simulink model "ASM_Traffic"  (R2026a)
settings: Solver=ode1  StartTime=SIM.tstart.v  StopTime=SIM.tend.v  FixedStep=SIM.StepSize.v
PostLoadFcn:
  | if any(exist('dsrtsu_mdlpostloadfcn', 'file') ~= 0), dsrtsu_mdlpostloadfcn('Execute', bdroot); end
  | try, asm_mdl_postloadfcn(bdroot, 'UpdateModel', 3600); catch, disp(lasterr); end,
InitFcn:
  | , if any(exist('rtifpga_mdlclblib', 'file') ~= 0), rtifpga_mdlclblib('Init', bdroot); end,
  | , if any(exist('dsmpb_private', 'file') ~= 0), dsmpb_private('dsmpb_mdlclblib', 'Init', bdroot); end,
model workspace (MAT data in the model file):
  asmReferencePath = [0 0.01 0.02 0.03 0.04 0.05 0.06 0.07 0.08 0.09 0.1 0.11 ... (350007 elements, 50001x7)]
  roadBounds : Simulink.Parameter (value not decoded)
  safetyAxes : Simulink.Parameter (value not decoded)
undefined symbols (not defined in the file): _to_, a0b2, ASM_BrakeHydraulics_DemoSystems, ASM_VehicleDynamics_DemoSystems, b98103fe8ad365046cd0, BrakeCircuit, controllerConfig, CPT, Crankshaft, DiscIntNeverNeededParam, dsmsi, FinalDriveAssembly, MDL, ModeSignals, mu, Pos_BrakePedal_Maneuver, rad, RefSignals, roadFamilyData, roadFamilyId, s_to_rpm, SIM, SoftECU, Suspension, Tire, Transmission
libraries: ASM_Traffic_lib x135, simulink x98, ASM_Utils_lib x77, ASM_VehicleDynamics_lib x70, ASM_Environment_lib x22, dsmpblib x20, dsmsilib x15, MDLD_Utils_lib x10, ASM_BrakeHydraulics_lib x3, sl_discontinuities x2
(part 23 of 65)

== system ASM_Traffic/Drivetrain/Plant/Drivetrain/Transmission ==
  n_Engine[rad|s] : Inport
  Reset[0|1] : Inport  Port=2
  Trq_Engine[Nm] : Inport  Port=3
  Mode_Transmission[1|2] : Inport  Port=4
  Pos_ClutchPedal_MT[%] : Inport  Port=5
  Gear_MT[] : Inport  Port=6
  Enable_v_Init[0|1] : Inport  Port=7
  ECU_Signals : Inport  Port=8
  omega_In_Diff[rad|s] : Inport  Port=9
  ASMSignalCollector : Subsystem
  AutomaticActive : simulink/Logic and Bit Operations/Compare To Constant  relop===  const=2  OutDataTypeStr=boolean
  AutomaticTransmission : Subsystem  TreatAsAtomicUnit=on
  Bus Selector2 : BusSelector  OutputSignals=Ctrl_Lockup_Clutch[0_1],Gear[]
  Dummy : Constant  Value=0
  Goto Tag Visibility1 : GotoTagVisibility  GotoTag=ASMBUS_ManualTransmission
  Goto Tag Visibility2 : GotoTagVisibility  GotoTag=ASMBUS_AutomaticTransmission
  ManualActive : simulink/Logic and Bit Operations/Compare To Constant  relop===  const=1  OutDataTypeStr=boolean
  ManualTransmission : Subsystem  TreatAsAtomicUnit=on
  Multiport Switch : MultiPortSwitch  Inputs=2  InputSameDT=off
  Multiport Switch1 : MultiPortSwitch  Inputs=2  InputSameDT=off
  Multiport Switch2 : MultiPortSwitch  Inputs=2  InputSameDT=off
  Sat_TrmMode : Saturate  UpperLimit=2  LowerLimit=1
  Terminator : Terminator
  Trq_Fric[Nm] : Outport  VectorParamsAs1DForOutWhenUnconnected=off
  omega_In_Trm[rad|s] : Outport  Port=2  VectorParamsAs1DForOutWhenUnconnected=off
  Inertia_Out_Trm[kgm2] : Outport  Port=3  VectorParamsAs1DForOutWhenUnconnected=off
  Trq_Out_Trm[Nm] : Outport  Port=4  VectorParamsAs1DForOutWhenUnconnected=off
  tag scope: ASMBUS_AutomaticTransmission=scoped, ASMBUS_ManualTransmission=scoped
  wires:
  AutomaticTransmission/3(omega_In_Trm[rad|s]) -> Multiport Switch2/3
  Multiport Switch2/1 -> omega_In_Trm[rad|s]/1
  ManualTransmission/3(omega_In_Trm[rad|s]) -> Multiport Switch2/2
  Enable_v_Init[0|1]/1 -> ManualTransmission/6(Enable_v_Init[0|1]), AutomaticTransmission/6(Enable_v_Init[0|1])
  n_Engine[rad|s]/1 -> ManualTransmission/3(n_Engine[rad|s]), AutomaticTransmission/3(n_Engine[rad|s])
  ECU_Signals/1 -> Bus Selector2/1
  ManualTransmission/1(ASMSignalBus) -> [ASMBUS_ManualTransmission]
  AutomaticTransmission/1(ASMSignalBus) -> [ASMBUS_AutomaticTransmission]
  Bus Selector2/2 -> ASMSignalCollector/3(Gear_AT[]), AutomaticTransmission/2(Gear[])  "<Gear[]>"
  Bus Selector2/1 -> AutomaticTransmission/1(Ctrl_Lockup_Clutch[0_1])  "<Ctrl_Lockup_Clutch[0_1]>"
  Sat_TrmMode/1 -> AutomaticActive/1, ManualActive/1, Multiport Switch/1, Multiport Switch1/1, ASMSignalCollector/1(Mode_Transmission[1|2]), Multiport Switch2/1
  ManualActive/1 -> ManualTransmission/Enable
  Trq_Engine[Nm]/1 -> Terminator/1
  Reset[0|1]/1 -> ManualTransmission/5(Reset[0|1]), AutomaticTransmission/5(Reset[0|1])
  AutomaticTransmission/4(Trq_Out_Trm[Nm]) -> Multiport Switch1/3
  AutomaticTransmission/2(Trq_In_Converter[Nm]) -> Multiport Switch/3
  Multiport Switch1/1 -> Trq_Out_Trm[Nm]/1
  Multiport Switch/1 -> Trq_Fric[Nm]/1
  Dummy/1 -> Inertia_Out_Trm[kgm2]/1
  ManualTransmission/2(Trq_Fric[Nm]) -> Multiport Switch/2
  ManualTransmission/4(Trq_Out_Trm[Nm]) -> Multiport Switch1/2
  Mode_Transmission[1|2]/1 -> Sat_TrmMode/1
  Pos_ClutchPedal_MT[%]/1 -> ManualTransmission/1(Pos_ClutchPedal[%])
  Gear_MT[]/1 -> ASMSignalCollector/2(Gear_MT[]), ManualTransmission/2(Gear[])
  omega_In_Diff[rad|s]/1 -> ManualTransmission/4(omega_In_Diff[rad|s]), AutomaticTransmission/4(omega_In_Diff[rad|s])
  AutomaticActive/1 -> AutomaticTransmission/Enable

== system ASM_Traffic/Drivetrain/Plant/UserInterface/ASMSignalBus_Plant ==
  In : Inport
  Terminator_1 : Terminator
  tag scope: ASMBUS_Drivetrain_Plant=global
  wires:
  In/1 -> [ASMBUS_Drivetrain_Plant]  "Plant"
  [ASMBUS_Drivetrain_Plant] -> Terminator_1/1

== system ASM_Traffic/Drivetrain/Plant/UserInterface/DISP_Plant ==
  In : Inport
  ActiveTransmission : Subsystem
  AutomaticTransmission : Subsystem
  Bus Selector2 : BusSelector  OutputSignals=Crankshaft,Starter,FinalDriveAssembly.Shaft_CF.Trq_CF_Shaft[Nm],FinalDriveAssembly.Shaft_CR.Trq_CR_Shaft[Nm],FinalDriveAssembly.Shaft_FL.Trq_FL_Shaft[Nm],FinalDriveAssembly.Shaft_FR.Trq_FR_Shaft[Nm],FinalDriveAssembly.Shaft_RL.Trq_RL_Shaft[Nm],FinalDriveAssembly.Shaft_RR.Trq_RR_Shaft[Nm],Transmission.OutputSignals,Transmission.Manual,Transmission.Automatic
  EngineSpeed : Subsystem
  ManualTransmission : Subsystem
  Shafts : Subsystem
  wires:
  In/1 -> Bus Selector2/1
  Bus Selector2/7 -> Shafts/5(Shaft_RL)  "<Trq_RL_Shaft[Nm]>"
  Bus Selector2/1 -> EngineSpeed/1(Crankshaft)  "<Crankshaft>"
  Bus Selector2/10 -> ManualTransmission/1(ManTrm)  "<Manual>"
  Bus Selector2/2 -> EngineSpeed/2(Starter)  "<Starter>"
  Bus Selector2/4 -> Shafts/2(Shaft_CR)  "<Trq_CR_Shaft[Nm]>"
  Bus Selector2/3 -> Shafts/1(Shaft_CF)  "<Trq_CF_Shaft[Nm]>"
  Bus Selector2/9 -> ActiveTransmission/1(ActiveTrm)  "<OutputSignals>"
  Bus Selector2/6 -> Shafts/4(Shaft_FR)  "<Trq_FR_Shaft[Nm]>"
  Bus Selector2/5 -> Shafts/3(Shaft_FL)  "<Trq_FL_Shaft[Nm]>"
  Bus Selector2/8 -> Shafts/6(Shaft_RR)  "<Trq_RR_Shaft[Nm]>"
  Bus Selector2/11 -> AutomaticTransmission/1(AutoTrm)  "<Automatic>"

== system ASM_Traffic/Drivetrain/Plant/UserInterface/PAR_Plant ==
  Bus Creator1 : BusCreator  Inputs=5
  Const_LoadTorque[Nm] : Constant  Value=0
  DRIVETRAIN_VARIANT_SWITCHES : ASM_VehicleDynamics_lib/Drivetrain/DRIVETRAIN_VARIANT_SWITCHES  Tag=ASM_SUBCOMPONENT  SW_Transmission_Mode=MDL.Drivetrain.SW_Transmission_Mode.v  SW_Drivetrain_Mode=MDL.Drivetrain.SW_Drivetrain_Mode.v  ASMProperties=struct('Name','DRIVETRAIN_VARIANT_SWITCHES','Version','5.0','Library','ASM_VehicleDynamics_lib')  ASMInstanceName=drivetrain_variant_switches  ASMInstanceID=1
  ModelDesk_MC_ID_Drivetrain : ASM_Utils_lib/ModelDeskInterface/ModelDesk_MC  Tag=ASM_MAINCOMPONENT  Editable=off  MainComponent=Drivetrain
  Sw_CrankShaft_Reset[0Disabled|1Enabled] : Constant
  Sw_LoadTorque[0Clutch|1Constant] : Constant  Value=0
  Out : Outport  VectorParamsAs1DForOutWhenUnconnected=off
  wires:
  Sw_LoadTorque[0Clutch|1Constant]/1 -> Bus Creator1/3  "Sw_LoadTorque[0Clutch|1Constant]"
  Const_LoadTorque[Nm]/1 -> Bus Creator1/4  "Const_LoadTorque[Nm]"
  Sw_CrankShaft_Reset[0Disabled|1Enabled]/1 -> Bus Creator1/5  "Sw_CrankShaft_Reset[0Disabled|1Enabled]"
  DRIVETRAIN_VARIANT_SWITCHES/2 -> Bus Creator1/2  "Mode_Drivetrain[1AWD|2FWD|3RWD|4FF-4WD|5FF]"
  Bus Creator1/1 -> Out/1  "UserInterface"
  DRIVETRAIN_VARIANT_SWITCHES/1 -> Bus Creator1/1  "Mode_Transmission[1Manual|2Automatic]"

== system ASM_Traffic/Drivetrain/SignalInterface/ASMSignalInterface/signal_structure ==
  ASMSignalBus : Inport
  Automatic : BusSelector  OutputSignals=LockUpClutch,GearBox,TorqueConverter
  BusSelector_1 : BusSelector  OutputSignals=Control,Plant
  CentralDifferential : BusSelector  OutputSignals=omega_Cage[rad|s],omega_In_CentralDiff[rad|s],Shaft_CF,Shaft_CR,Trq_Lock[Nm],omega_Out_Front_CentralDiff[rad|s],omega_Out_Rear_CentralDiff[rad|s],Const_i_MainReductionGear[],Const_TrqDistribution[]
  Clutch : BusSelector  OutputSignals=Trq_Fric_Clutch[Nm],omega_delta_Clutch[rad|s],omega_Out_ClutchPlate[rad|s],Trq_TorsionSpring_Clutch[Nm]
  Clutch_4WD : BusSelector  OutputSignals=omega_Clutch_4WD_In[rad|s],Trq_Lock_Clutch_4WD[Nm],omega_Clutch_4WD_Out[rad|s]
  ContentID : Constant  Value=632359247
  Control : BusSelector  OutputSignals=Lockup_Clutch_Control,Shift_Lock_Control,Shift_Strategy,Tip_Shift_Control,Torque_Intervention_Control
  Crankshaft : BusSelector  OutputSignals=Trq_Mass_Mod[Nm],Const_Inertia_Engine[kgm2],Trq_Eff_Crank[Nm],n_Engine[rad|s],n_Engine[rpm]
  FinalDriveAssembly : BusSelector  OutputSignals=i_FrontDrive[],i_RearDrive[],TrqDistri_Front_Rear[0_1],i_FinalDrive[],CentralDifferential,FrontDifferential,RearDifferential,Shaft_TGCL4WD,Shaft_CF,Shaft_CR,TransferGearbox,Clutch_4WD,Shaft_FL,Shaft_FR,Shaft_RL,Shaft_RR,Trq_Out_Front_Diff[Nm],Trq_Shaft[FL;FR;RL;RR][Nm]
  FrontDifferential : BusSelector  OutputSignals=omega_Cage[rad|s],omega_In_FrontDifferential[rad|s],Shaft_FL,Shaft_FR,Trq_Lock_FrontDifferential[Nm],omega_Out_Left_FrontDifferential[rad|s],omega_Out_Right_FrontDifferential[rad|s],Const_i_MainReductionGear[],Const_TrqDistribution[]
  GearBox : BusSelector  OutputSignals=i_unsync_Trm[],i_Trm[],Trq_Out_Trm[Nm],omega_In_Trm[rad|s],omega_Out_Trm[rad|s],Inertia_Trm[kgm2]
  GearBox1 : BusSelector  OutputSignals=i_unsync_Trm[],i_Trm[],Trq_Out_Trm[Nm],omega_In_Trm[rad|s],omega_Out_Trm[rad|s],Inertia_Trm[kgm2]
  InfoBlock : Subsystem
      mask Display: fprintf('Structural changes of the signal bus require an update \nof the ''ASMSignalCollector'' block. \n\nTo start the update process double click the parent block.\n\n WARNING:\n During update this subsystem will be cleared completely')
  LockUpClutch : BusSelector  OutputSignals=Trq_Fric_Clutch[Nm],omega_delta_Clutch[rad|s],omega_Out_ClutchPlate[rad|s],Trq_TorsionSpring_Clutch[Nm]
  Lockup_Clutch_Control : BusSelector  OutputSignals=Ctrl_Lockup_Clutch[0_1]
  MDLD_DATA_CAPTURE : MDLD_Utils_lib/ModelDeskPlotInterface/DataCapture_Sfcn/MDLD_DATA_CAPTURE  inputPortWidth=94  measurementSignals=[0 0 0 0 0 0 0 0 0 0 0 0 0 0 0 0 0 0 0 0 0 0 0 0 0 0 0 0 0 0 0 0 0 0 0 0 0 0 0 0 0 0 0 0 0 0 0 0 0 0 0 0 0 0 0 0 0 0 0 0 0 0 0 0 0 0 0 0 0 0 0 0 0 0 0 0 0 0 0 0 0 0 0 0 0 0 0 0 0 0 0 0 0 0]  downsampling=1  samplingPeriod=SIM.StepSize.v  uuid=0  ASMProperties=struct('Name','mdld_data_capture','Version','1.0','Library','mdld_utils_lib')  startTriggerDelay=0  startTriggerLogic=0  startTriggerCount=0  startTriggerConditions=[0,0,0,0,0,0,0,0,0]  stopTriggerDelay=0  stopTriggerLogic=0  stopTriggerCount=0  stopTriggerConditions=[0,0,0,0,0,0,0,0,0]  ContentID_RefStruct=632359247
  Manual : BusSelector  OutputSignals=Clutch,GearBox
  OutputSignals : BusSelector  OutputSignals=i_unsync_Trm[],i_Trm[],Trq_Out_Trm[Nm],omega_In_Trm[rad|s],Inertia_Trm[kgm2],omega_Out_Trm[rad|s],Gear[]
  Plant : BusSelector  OutputSignals=Crankshaft,Starter,TestBench,Transmission,FinalDriveAssembly,Type_Engine_1[0Unkown|1Other|2Otto|3Diesel|4Electric],Trq_MeanEff_Engine[Nm]
  RearDifferential : BusSelector  OutputSignals=omega_Cage[rad|s],omega_In_RearDifferential[rad|s],Shaft_RL,Shaft_RR,Trq_Lock_RearDifferential[Nm],omega_Out_Left_RearDifferential[rad|s],omega_Out_Right_RearDifferential[rad|s],Const_i_MainReductionGear[],Const_TrqDistribution[]
  Reshape_89 : Reshape
  Shaft_CF : BusSelector  OutputSignals=Trq_CF_Shaft[Nm]
  Shaft_CF1 : BusSelector  OutputSignals=Trq_CF_Shaft[Nm]
  Shaft_CR : BusSelector  OutputSignals=Trq_CR_Shaft[Nm]
  Shaft_CR1 : BusSelector  OutputSignals=Trq_CR_Shaft[Nm]
  Shaft_FL : BusSelector  OutputSignals=Trq_FL_Shaft[Nm]
  Shaft_FL1 : BusSelector  OutputSignals=Trq_FL_Shaft[Nm]
  Shaft_FR : BusSelector  OutputSignals=Trq_FR_Shaft[Nm]
  Shaft_FR1 : BusSelector  OutputSignals=Trq_FR_Shaft[Nm]
  Shaft_RL : BusSelector  OutputSignals=Trq_RL_Shaft[Nm]
  Shaft_RL1 : BusSelector  OutputSignals=Trq_RL_Shaft[Nm]
  Shaft_RR : BusSelector  OutputSignals=Trq_RR_Shaft[Nm]
  Shaft_RR1 : BusSelector  OutputSignals=Trq_RR_Shaft[Nm]
  Shaft_TGCL4WD : BusSelector  OutputSignals=Trq_TGCL4WD_Shaft[Nm]
  Shift_Lock_Control : BusSelector  OutputSignals=Ctrl_Parking_Pawl[0|1]
  Shift_Strategy : BusSelector  OutputSignals=Gear_Requested[]
  SignalFilter : Mux  Inputs=91
  SignalFilterGain : Gain
  Starter : BusSelector  OutputSignals=Trq_Starter[Nm],Inertia_Starter[kgm2]
  Terminator : Terminator
  TestBench : BusSelector  OutputSignals=Trq_TestBench[Nm],Inertia_TestBench[kgm2]
  Tip_Shift_Control : BusSelector  OutputSignals=Gear_Requested[]
  TorqueConverter : BusSelector  OutputSignals=Trq_Pump[Nm],Trq_Turbine[Nm]
  Torque_Intervention_Control : BusSelector  OutputSignals=Factor_Trq_Engine_Red[%],Gear[]
  TransferGearbox : BusSelector  OutputSignals=Trq_Cage[Nm],omega_Shaft[rad|s]
  Transmission : BusSelector  OutputSignals=Manual,Automatic,OutputSignals
  wires:
  ASMSignalBus/1 -> BusSelector_1/1
  BusSelector_1/1 -> Control/1  "<Control>"
  Control/1 -> Lockup_Clutch_Control/1  "<Lockup_Clutch_Control>"
  Control/2 -> Shift_Lock_Control/1  "<Shift_Lock_Control>"
  Control/3 -> Shift_Strategy/1  "<Shift_Strategy>"
  Control/4 -> Tip_Shift_Control/1  "<Tip_Shift_Control>"
  Control/5 -> Torque_Intervention_Control/1  "<Torque_Intervention_Control>"
  BusSelector_1/2 -> Plant/1  "<Plant>"
  Plant/1 -> Crankshaft/1  "<Crankshaft>"
  Plant/2 -> Starter/1  "<Starter>"
  Plant/3 -> TestBench/1  "<TestBench>"
  Plant/4 -> Transmission/1  "<Transmission>"
  Transmission/1 -> Manual/1  "<Manual>"
  Manual/1 -> Clutch/1  "<Clutch>"
  Manual/2 -> GearBox/1  "<GearBox>"
  Transmission/2 -> Automatic/1  "<Automatic>"
  Automatic/1 -> LockUpClutch/1  "<LockUpClutch>"
  Automatic/2 -> GearBox1/1  "<GearBox>"
  Automatic/3 -> TorqueConverter/1  "<TorqueConverter>"
  Transmission/3 -> OutputSignals/1  "<OutputSignals>"
  Plant/5 -> FinalDriveAssembly/1  "<FinalDriveAssembly>"
  FinalDriveAssembly/5 -> CentralDifferential/1  "<CentralDifferential>"
  CentralDifferential/3 -> Shaft_CF/1  "<Shaft_CF>"
  CentralDifferential/4 -> Shaft_CR/1  "<Shaft_CR>"
  FinalDriveAssembly/6 -> FrontDifferential/1  "<FrontDifferential>"
  FrontDifferential/3 -> Shaft_FL/1  "<Shaft_FL>"
  FrontDifferential/4 -> Shaft_FR/1  "<Shaft_FR>"
  FinalDriveAssembly/7 -> RearDifferential/1  "<RearDifferential>"
  RearDifferential/3 -> Shaft_RL/1  "<Shaft_RL>"
  RearDifferential/4 -> Shaft_RR/1  "<Shaft_RR>"
  FinalDriveAssembly/8 -> Shaft_TGCL4WD/1  "<Shaft_TGCL4WD>"
  FinalDriveAssembly/9 -> Shaft_CF1/1  "<Shaft_CF>"
  FinalDriveAssembly/10 -> Shaft_CR1/1  "<Shaft_CR>"
  FinalDriveAssembly/11 -> TransferGearbox/1  "<TransferGearbox>"
  FinalDriveAssembly/12 -> Clutch_4WD/1  "<Clutch_4WD>"
  FinalDriveAssembly/13 -> Shaft_FL1/1  "<Shaft_FL>"
  FinalDriveAssembly/14 -> Shaft_FR1/1  "<Shaft_FR>"
  FinalDriveAssembly/15 -> Shaft_RL1/1  "<Shaft_RL>"
  FinalDriveAssembly/16 -> Shaft_RR1/1  "<Shaft_RR>"
  ContentID/1 -> Terminator/1
  Lockup_Clutch_Control/1 -> SignalFilter/1  "<Ctrl_Lockup_Clutch[0_1]>"
  Shift_Lock_Control/1 -> SignalFilter/2  "<Ctrl_Parking_Pawl[0|1]>"
  Shift_Strategy/1 -> SignalFilter/3  "<Gear_Requested[]>"
  Tip_Shift_Control/1 -> SignalFilter/4  "<Gear_Requested[]>"
  Torque_Intervention_Control/1 -> SignalFilter/5  "<Factor_Trq_Engine_Red[%]>"
  Torque_Intervention_Control/2 -> SignalFilter/6  "<Gear[]>"
  Crankshaft/1 -> SignalFilter/7  "<Trq_Mass_Mod[Nm]>"
  Crankshaft/2 -> SignalFilter/8  "<Const_Inertia_Engine[kgm2]>"
  Crankshaft/3 -> SignalFilter/9  "<Trq_Eff_Crank[Nm]>"
  Crankshaft/4 -> SignalFilter/10  "<n_Engine[rad|s]>"
  Crankshaft/5 -> SignalFilter/11  "<n_Engine[rpm]>"
  Starter/1 -> SignalFilter/12  "<Trq_Starter[Nm]>"
  Starter/2 -> SignalFilter/13  "<Inertia_Starter[kgm2]>"
  TestBench/1 -> SignalFilter/14  "<Trq_TestBench[Nm]>"
  TestBench/2 -> SignalFilter/15  "<Inertia_TestBench[kgm2]>"
  Clutch/1 -> SignalFilter/16  "<Trq_Fric_Clutch[Nm]>"
  Clutch/2 -> SignalFilter/17  "<omega_delta_Clutch[rad|s]>"
  Clutch/3 -> SignalFilter/18  "<omega_Out_ClutchPlate[rad|s]>"
  Clutch/4 -> SignalFilter/19  "<Trq_TorsionSpring_Clutch[Nm]>"
  GearBox/1 -> SignalFilter/20  "<i_unsync_Trm[]>"
  GearBox/2 -> SignalFilter/21  "<i_Trm[]>"
  GearBox/3 -> SignalFilter/22  "<Trq_Out_Trm[Nm]>"
  GearBox/4 -> SignalFilter/23  "<omega_In_Trm[rad|s]>"
  GearBox/5 -> SignalFilter/24  "<omega_Out_Trm[rad|s]>"
  GearBox/6 -> SignalFilter/25  "<Inertia_Trm[kgm2]>"
  LockUpClutch/1 -> SignalFilter/26  "<Trq_Fric_Clutch[Nm]>"
  LockUpClutch/2 -> SignalFilter/27  "<omega_delta_Clutch[rad|s]>"
  LockUpClutch/3 -> SignalFilter/28  "<omega_Out_ClutchPlate[rad|s]>"
  LockUpClutch/4 -> SignalFilter/29  "<Trq_TorsionSpring_Clutch[Nm]>"
  GearBox1/1 -> SignalFilter/30  "<i_unsync_Trm[]>"
  GearBox1/2 -> SignalFilter/31  "<i_Trm[]>"
  GearBox1/3 -> SignalFilter/32  "<Trq_Out_Trm[Nm]>"
  GearBox1/4 -> SignalFilter/33  "<omega_In_Trm[rad|s]>"
  GearBox1/5 -> SignalFilter/34  "<omega_Out_Trm[rad|s]>"
  GearBox1/6 -> SignalFilter/35  "<Inertia_Trm[kgm2]>"
  TorqueConverter/1 -> SignalFilter/36  "<Trq_Pump[Nm]>"
  TorqueConverter/2 -> SignalFilter/37  "<Trq_Turbine[Nm]>"
  OutputSignals/1 -> SignalFilter/38  "<i_unsync_Trm[]>"
  OutputSignals/2 -> SignalFilter/39  "<i_Trm[]>"
  OutputSignals/3 -> SignalFilter/40  "<Trq_Out_Trm[Nm]>"
  OutputSignals/4 -> SignalFilter/41  "<omega_In_Trm[rad|s]>"
  OutputSignals/5 -> SignalFilter/42  "<Inertia_Trm[kgm2]>"
  OutputSignals/6 -> SignalFilter/43  "<omega_Out_Trm[rad|s]>"
  OutputSignals/7 -> SignalFilter/44  "<Gear[]>"
  FinalDriveAssembly/1 -> SignalFilter/45  "<i_FrontDrive[]>"
  FinalDriveAssembly/2 -> SignalFilter/46  "<i_RearDrive[]>"
  FinalDriveAssembly/3 -> SignalFilter/47  "<TrqDistri_Front_Rear[0_1]>"
  FinalDriveAssembly/4 -> SignalFilter/48  "<i_FinalDrive[]>"
  CentralDifferential/1 -> SignalFilter/49  "<omega_Cage[rad|s]>"
  CentralDifferential/2 -> SignalFilter/50  "<omega_In_CentralDiff[rad|s]>"
  Shaft_CF/1 -> SignalFilter/51  "<Trq_CF_Shaft[Nm]>"
  Shaft_CR/1 -> SignalFilter/52  "<Trq_CR_Shaft[Nm]>"
  CentralDifferential/5 -> SignalFilter/53  "<Trq_Lock[Nm]>"
  CentralDifferential/6 -> SignalFilter/54  "<omega_Out_Front_CentralDiff[rad|s]>"
  CentralDifferential/7 -> SignalFilter/55  "<omega_Out_Rear_CentralDiff[rad|s]>"
  CentralDifferential/8 -> SignalFilter/56  "<Const_i_MainReductionGear[]>"
  CentralDifferential/9 -> SignalFilter/57  "<Const_TrqDistribution[]>"
  FrontDifferential/1 -> SignalFilter/58  "<omega_Cage[rad|s]>"
  FrontDifferential/2 -> SignalFilter/59  "<omega_In_FrontDifferential[rad|s]>"
  Shaft_FL/1 -> SignalFilter/60  "<Trq_FL_Shaft[Nm]>"
  Shaft_FR/1 -> SignalFilter/61  "<Trq_FR_Shaft[Nm]>"
  FrontDifferential/5 -> SignalFilter/62  "<Trq_Lock_FrontDifferential[Nm]>"
  FrontDifferential/6 -> SignalFilter/63  "<omega_Out_Left_FrontDifferential[rad|s]>"
  FrontDifferential/7 -> SignalFilter/64  "<omega_Out_Right_FrontDifferential[rad|s]>"
  FrontDifferential/8 -> SignalFilter/65  "<Const_i_MainReductionGear[]>"
  FrontDifferential/9 -> SignalFilter/66  "<Const_TrqDistribution[]>"
  RearDifferential/1 -> SignalFilter/67  "<omega_Cage[rad|s]>"
  RearDifferential/2 -> SignalFilter/68  "<omega_In_RearDifferential[rad|s]>"
  Shaft_RL/1 -> SignalFilter/69  "<Trq_RL_Shaft[Nm]>"
  Shaft_RR/1 -> SignalFilter/70  "<Trq_RR_Shaft[Nm]>"
  RearDifferential/5 -> SignalFilter/71  "<Trq_Lock_RearDifferential[Nm]>"
  RearDifferential/6 -> SignalFilter/72  "<omega_Out_Left_RearDifferential[rad|s]>"
  RearDifferential/7 -> SignalFilter/73  "<omega_Out_Right_RearDifferential[rad|s]>"
  RearDifferential/8 -> SignalFilter/74  "<Const_i_MainReductionGear[]>"
  RearDifferential/9 -> SignalFilter/75  "<Const_TrqDistribution[]>"
  Shaft_TGCL4WD/1 -> SignalFilter/76  "<Trq_TGCL4WD_Shaft[Nm]>"
  Shaft_CF1/1 -> SignalFilter/77  "<Trq_CF_Shaft[Nm]>"
  Shaft_CR1/1 -> SignalFilter/78  "<Trq_CR_Shaft[Nm]>"
  TransferGearbox/1 -> SignalFilter/79  "<Trq_Cage[Nm]>"
  TransferGearbox/2 -> SignalFilter/80  "<omega_Shaft[rad|s]>"
  Clutch_4WD/1 -> SignalFilter/81  "<omega_Clutch_4WD_In[rad|s]>"
  Clutch_4WD/2 -> SignalFilter/82  "<Trq_Lock_Clutch_4WD[Nm]>"
  Clutch_4WD/3 -> SignalFilter/83  "<omega_Clutch_4WD_Out[rad|s]>"
  Shaft_FL1/1 -> SignalFilter/84  "<Trq_FL_Shaft[Nm]>"
  Shaft_FR1/1 -> SignalFilter/85  "<Trq_FR_Shaft[Nm]>"
  Shaft_RL1/1 -> SignalFilter/86  "<Trq_RL_Shaft[Nm]>"
  Shaft_RR1/1 -> SignalFilter/87  "<Trq_RR_Shaft[Nm]>"
  FinalDriveAssembly/17 -> SignalFilter/88  "<Trq_Out_Front_Diff[Nm]>"
  FinalDriveAssembly/18 -> Reshape_89/1  "<Trq_Shaft[FL;FR;RL;RR][Nm]>"
  Reshape_89/1 -> SignalFilter/89
  Plant/6 -> SignalFilter/90  "<Type_Engine_1[0Unkown|1Other|2Otto|3Diesel|4Electric]>"
  Plant/7 -> SignalFilter/91  "<Trq_MeanEff_Engine[Nm]>"
  SignalFilter/1 -> SignalFilterGain/1
  SignalFilterGain/1 -> MDLD_DATA_CAPTURE/1

== system ASM_Traffic/Drivetrain/SignalInterface/ExternalOutports/Select_Outport_Signals ==
  ASMSignalBus : Inport
  Bus Selector : BusSelector  OutputSignals=Crankshaft.n_Engine[rpm],Crankshaft.Trq_Eff_Crank[Nm]  OutputAsBus=on
  Bus Selector1 : BusSelector  OutputSignals=Starter,TestBench
  Bus Selector2 : BusSelector  OutputSignals=Transmission.OutputSignals.i_Trm[],Transmission.OutputSignals.Trq_Out_Trm[Nm],Transmission.OutputSignals.omega_In_Trm[rad|s],Transmission.OutputSignals.omega_Out_Trm[rad|s],Transmission.OutputSignals.Gear[],Transmission.OutputSignals.i_unsync_Trm[]  OutputAsBus=on
  Bus Selector3 : BusSelector  OutputSignals=FinalDriveAssembly
  Crankshaft : Outport  VectorParamsAs1DForOutWhenUnconnected=off
  Starter : Outport  Port=2  VectorParamsAs1DForOutWhenUnconnected=off
  TestBench : Outport  Port=3  VectorParamsAs1DForOutWhenUnconnected=off
  Transmission : Outport  Port=4  VectorParamsAs1DForOutWhenUnconnected=off
  FinalDriveAssembly : Outport  Port=5  VectorParamsAs1DForOutWhenUnconnected=off
  wires:
  ASMSignalBus/1 -> Bus Selector3/1, Bus Selector2/1, Bus Selector1/1, Bus Selector/1
  Bus Selector/1 -> Crankshaft/1
  Bus Selector1/1 -> Starter/1  "<Starter>"
  Bus Selector1/2 -> TestBench/1  "<TestBench>"
  Bus Selector2/1 -> Transmission/1
  Bus Selector3/1 -> FinalDriveAssembly/1  "<FinalDriveAssembly>"

== system ASM_Traffic/ElectricalSystem/Control/UserInterface/ASMSignalBus_Control ==
  In : Inport
  Terminator_1 : Terminator
  tag scope: ASMBUS_ElectricalSystem_Control=global
  wires:
  In/1 -> [ASMBUS_ElectricalSystem_Control]  "Control"
  [ASMBUS_ElectricalSystem_Control] -> Terminator_1/1

== system ASM_Traffic/ElectricalSystem/Control/UserInterface/DISP_Control ==
  In : Inport
  Terminator : Terminator
  wires:
  In/1 -> Terminator/1

== system ASM_Traffic/ElectricalSystem/Control/UserInterface/PAR_Control ==
  Constant : Constant  Value=0
  Out : Outport  VectorParamsAs1DForOutWhenUnconnected=off
  wires:
  Constant/1 -> Out/1

== system ASM_Traffic/ElectricalSystem/Interface_In/ModelSignals/Sw_ModelDeskPlottingInterface[0Disabled|1Enabled]_ ==
  In1 : Inport
  Gain : Gain
  Out1 : Outport
  wires:
  Gain/1 -> Out1/1
  In1/1 -> Gain/1

== system ASM_Traffic/ElectricalSystem/Interface_In/ModelSignals/Sw_ModelPortBlocks[0Disabled|1Enabled]_ ==
  In1 : Inport
  Gain : Gain
  Out1 : Outport
  wires:
  Gain/1 -> Out1/1
  In1/1 -> Gain/1

== system ASM_Traffic/ElectricalSystem/Interface_Out/Control_ModelSignals/SOC_Estimated_Max[%]_ ==
  In1 : Inport
  Gain : Gain  SaturateOnIntegerOverflow=on  OutDataTypeStr=Inherit: Same as input  ParamDataTypeStr=Inherit: Same as input
  Out1 : Outport  VectorParamsAs1DForOutWhenUnconnected=off
  wires:
  Gain/1 -> Out1/1
  In1/1 -> Gain/1

== system ASM_Traffic/ElectricalSystem/Interface_Out/Control_ModelSignals/SOC_Estimated_Mean[%]_ ==
  In1 : Inport
  Gain : Gain  SaturateOnIntegerOverflow=on  OutDataTypeStr=Inherit: Same as input  ParamDataTypeStr=Inherit: Same as input
  Out1 : Outport  VectorParamsAs1DForOutWhenUnconnected=off
  wires:
  In1/1 -> Gain/1
  Gain/1 -> Out1/1

== system ASM_Traffic/ElectricalSystem/Interface_Out/Plant_ModelSignals/I_DCDC_LS[A]_ ==
  In1 : Inport
  Gain : Gain  SaturateOnIntegerOverflow=on  OutDataTypeStr=Inherit: Same as input  ParamDataTypeStr=Inherit: Same as input
  Out1 : Outport  VectorParamsAs1DForOutWhenUnconnected=off
  wires:
  In1/1 -> Gain/1
  Gain/1 -> Out1/1

== system ASM_Traffic/ElectricalSystem/Interface_Out/Plant_ModelSignals/I_DCLink[A]_ ==
  In1 : Inport
  Gain : Gain  SaturateOnIntegerOverflow=on  OutDataTypeStr=Inherit: Same as input  ParamDataTypeStr=Inherit: Same as input
  Out1 : Outport  VectorParamsAs1DForOutWhenUnconnected=off
  wires:
  In1/1 -> Gain/1
  Gain/1 -> Out1/1

== system ASM_Traffic/ElectricalSystem/Interface_Out/Plant_ModelSignals/SOC_Bat_LV[%]_ ==
  In1 : Inport
  Gain : Gain  SaturateOnIntegerOverflow=on  OutDataTypeStr=Inherit: Same as input  ParamDataTypeStr=Inherit: Same as input
  Out1 : Outport  VectorParamsAs1DForOutWhenUnconnected=off
  wires:
  In1/1 -> Gain/1
  Gain/1 -> Out1/1

== system ASM_Traffic/ElectricalSystem/Interface_Out/Plant_ModelSignals/State_DCLink[0Off|1On]_ ==
  In1 : Inport
  Gain : Gain  SaturateOnIntegerOverflow=on  OutDataTypeStr=Inherit: Same as input  ParamDataTypeStr=Inherit: Same as input
  Out1 : Outport  VectorParamsAs1DForOutWhenUnconnected=off
  wires:
  In1/1 -> Gain/1
  Gain/1 -> Out1/1

== system ASM_Traffic/ElectricalSystem/Interface_Out/Plant_ModelSignals/Sw_DCLink_Reset[0Disabled|1Enabled]_ ==
  In1 : Inport
  Gain : Gain  SaturateOnIntegerOverflow=on  OutDataTypeStr=Inherit: Same as input  ParamDataTypeStr=Inherit: Same as input
  Out1 : Outport  VectorParamsAs1DForOutWhenUnconnected=off
  wires:
  Gain/1 -> Out1/1
  In1/1 -> Gain/1

== system ASM_Traffic/ElectricalSystem/Interface_Out/Plant_ModelSignals/T_Bat_HV[degC]_ ==
  In1 : Inport
  Gain : Gain  SaturateOnIntegerOverflow=on  OutDataTypeStr=Inherit: Same as input  ParamDataTypeStr=Inherit: Same as input
  Out1 : Outport  VectorParamsAs1DForOutWhenUnconnected=off
  wires:
  In1/1 -> Gain/1
  Gain/1 -> Out1/1

== system ASM_Traffic/ElectricalSystem/Interface_Out/Plant_ModelSignals/T_Bat_LV[degC]_ ==
  In1 : Inport
  Gain : Gain  SaturateOnIntegerOverflow=on  OutDataTypeStr=Inherit: Same as input  ParamDataTypeStr=Inherit: Same as input
  Out1 : Outport  VectorParamsAs1DForOutWhenUnconnected=off
  wires:
  Gain/1 -> Out1/1
  In1/1 -> Gain/1

== system ASM_Traffic/ElectricalSystem/Interface_Out/Plant_ModelSignals/V_Bat_HV[V]_ ==
  In1 : Inport
  Gain : Gain  SaturateOnIntegerOverflow=on  OutDataTypeStr=Inherit: Same as input  ParamDataTypeStr=Inherit: Same as input
  Out1 : Outport  VectorParamsAs1DForOutWhenUnconnected=off
  wires:
  In1/1 -> Gain/1
  Gain/1 -> Out1/1

== system ASM_Traffic/ElectricalSystem/Interface_Out/Plant_ModelSignals/V_Bat_LV[V]_ ==
  In1 : Inport
  Gain : Gain  SaturateOnIntegerOverflow=on  OutDataTypeStr=Inherit: Same as input  ParamDataTypeStr=Inherit: Same as input
  Out1 : Outport  VectorParamsAs1DForOutWhenUnconnected=off
  wires:
  Gain/1 -> Out1/1
  In1/1 -> Gain/1

== system ASM_Traffic/ElectricalSystem/Interface_Out/Plant_ModelSignals/V_DCLink[V]_ ==
  In1 : Inport
  Gain : Gain  SaturateOnIntegerOverflow=on  OutDataTypeStr=Inherit: Same as input  ParamDataTypeStr=Inherit: Same as input
  Out1 : Outport  VectorParamsAs1DForOutWhenUnconnected=off
  wires:
  Gain/1 -> Out1/1
  In1/1 -> Gain/1

== system ASM_Traffic/ElectricalSystem/Plant/ElectricalSystemBasic/ASMSignalCollector ==
  BusCreator : BusCreator  Inputs=3
  ASMSignalBus : Outport  VectorParamsAs1DForOutWhenUnconnected=off
  wires:
  [ASMBUS_ElectricalSystem_DCLink] -> BusCreator/3
  [ASMBUS_ElectricalSystem_Battery_HV] -> BusCreator/2
  [ASMBUS_ElectricalSystem_Battery_LV] -> BusCreator/1
  BusCreator/1 -> ASMSignalBus/1  "Plant"

== system ASM_Traffic/ElectricalSystem/Plant/ElectricalSystemBasic/Battery_HV ==
  ASMSignalCollector : Subsystem
  Const_SOC_Bat[%] : Constant  Value=80
  Const_T_Bat[degC] : Constant  Value=25
  Const_V_Bat[V] : Constant  Value=48
  ASMSignalBus : Outport  VectorParamsAs1DForOutWhenUnconnected=off
  V_Bat[V] : Outport  Port=2  VectorParamsAs1DForOutWhenUnconnected=off
  SOC_Bat[%] : Outport  Port=3  VectorParamsAs1DForOutWhenUnconnected=off
  T_Bat[degC] : Outport  Port=4  VectorParamsAs1DForOutWhenUnconnected=off
  wires:
  ASMSignalCollector/1(ASMSignalBus) -> ASMSignalBus/1
  Const_V_Bat[V]/1 -> V_Bat[V]/1, ASMSignalCollector/1(V_Bat[V])
  Const_SOC_Bat[%]/1 -> ASMSignalCollector/2(SOC_Bat[%]), SOC_Bat[%]/1
  Const_T_Bat[degC]/1 -> T_Bat[degC]/1, ASMSignalCollector/3(T_Bat[degC])

== system ASM_Traffic/ElectricalSystem/Plant/ElectricalSystemBasic/Battery_LV ==
  ASMSignalCollector : Subsystem
  Const_SOC_Bat[%] : Constant  Value=80
  Const_T_Bat[degC] : Constant  Value=25
  Const_V_Bat[V] : Constant  Value=12
  ASMSignalBus : Outport  VectorParamsAs1DForOutWhenUnconnected=off
  V_Bat[V] : Outport  Port=2  VectorParamsAs1DForOutWhenUnconnected=off
  SOC_Bat[%] : Outport  Port=3  VectorParamsAs1DForOutWhenUnconnected=off
  T_Bat[degC] : Outport  Port=4  VectorParamsAs1DForOutWhenUnconnected=off
  wires:
  Const_T_Bat[degC]/1 -> ASMSignalCollector/3(T_Bat[degC]), T_Bat[degC]/1
  Const_SOC_Bat[%]/1 -> ASMSignalCollector/2(SOC_Bat[%]), SOC_Bat[%]/1
  Const_V_Bat[V]/1 -> ASMSignalCollector/1(V_Bat[V]), V_Bat[V]/1
  ASMSignalCollector/1(ASMSignalBus) -> ASMSignalBus/1

== system ASM_Traffic/ElectricalSystem/Plant/ElectricalSystemBasic/DCLink ==
  V_Bat[V] : Inport
  ASMSignalCollector : Subsystem
  ASMSignalBus : Outport  VectorParamsAs1DForOutWhenUnconnected=off
  V_DCLink[V] : Outport  Port=2  VectorParamsAs1DForOutWhenUnconnected=off
  wires:
  V_Bat[V]/1 -> ASMSignalCollector/1(V_DCLink[V]), V_DCLink[V]/1
  ASMSignalCollector/1(ASMSignalBus) -> ASMSignalBus/1

== system ASM_Traffic/ElectricalSystem/Plant/UserInterface/ASMSignalBus_Plant ==
  In : Inport
  Terminator_1 : Terminator
  tag scope: ASMBUS_ElectricalSystem_Plant=global
  wires:
  In/1 -> [ASMBUS_ElectricalSystem_Plant]  "Plant"
  [ASMBUS_ElectricalSystem_Plant] -> Terminator_1/1

== system ASM_Traffic/ElectricalSystem/Plant/UserInterface/DISP_Plant ==
  In : Inport
  Battery_HV : Scope  NumInputPorts=3
      settings: TimeSpan=5  ActiveDisplayYMinimum=-20  ActiveDisplayYMaximum=110  DataLoggingMaxPoints=20000  DataLoggingDecimation=10
  Battery_LV : Scope  NumInputPorts=3
      settings: TimeSpan=5  ActiveDisplayYMinimum=-20  ActiveDisplayYMaximum=110  DataLoggingMaxPoints=20000  DataLoggingDecimation=10  DataLoggingVariableName=ScopeData5
  Bus Selector1 : BusSelector  OutputSignals=Battery_LV.V_Bat[V],Battery_LV.SOC_Bat[%],Battery_LV.T_Bat[degC]
  Bus Selector2 : BusSelector  OutputSignals=Battery_HV.V_Bat[V],DCLink.V_DCLink[V],Battery_HV.SOC_Bat[%],Battery_HV.T_Bat[degC]
  Mux : Mux  Inputs=2
  SOC_HV[%] : Subsystem
      mask Display: disp('')
  SOC_LV[%] : Subsystem
      mask Display: disp('')
  T_Bat_HV[degC] : Subsystem
      mask Display: disp('')
  T_Bat_LV[degC] : Subsystem
      mask Display: disp('')
  V_Bat_HV[V] : Subsystem
      mask Display: disp('')
  V_Bat_LV[V] : Subsystem
      mask Display: disp('')
  V_DCLink[V] : Subsystem
      mask Display: disp('')
  wires:
  In/1 -> Bus Selector1/1, Bus Selector2/1
  V_Bat_LV[V]/1(Out1) -> Battery_LV/1  "V_Bat_LV[V]"
  Bus Selector1/1 -> V_Bat_LV[V]/1(In1)  "<V_Bat[V]>"
  Bus Selector1/2 -> SOC_LV[%]/1(In1)  "<SOC_Bat[%]>"
  Bus Selector1/3 -> T_Bat_LV[degC]/1(In1)  "<T_Bat[degC]>"
  SOC_LV[%]/1(Out1) -> Battery_LV/2  "SOC_LV[%]"
  T_Bat_LV[degC]/1(Out1) -> Battery_LV/3  "T_Bat_LV[degC]"
  T_Bat_HV[degC]/1(Out1) -> Battery_HV/3  "T_Bat_HV[degC]"
  SOC_HV[%]/1(Out1) -> Battery_HV/2  "SOC_HV[%]"
  Bus Selector2/4 -> T_Bat_HV[degC]/1(In1)  "<T_Bat[degC]>"
  Bus Selector2/3 -> SOC_HV[%]/1(In1)  "<SOC_Bat[%]>"
  Bus Selector2/1 -> V_Bat_HV[V]/1(In1)  "<V_Bat[V]>"
  V_Bat_HV[V]/1(Out1) -> Mux/1  "V_Bat_HV[V]"
  Bus Selector2/2 -> V_DCLink[V]/1(In1)  "<V_DCLink[V]>"
  Mux/1 -> Battery_HV/1  "V_HV[V]"
  V_DCLink[V]/1(Out1) -> Mux/2  "V_DCLink[V]"

== system ASM_Traffic/ElectricalSystem/Plant/UserInterface/PAR_Plant ==
  Ground : Constant  Value=0
  Out : Outport  VectorParamsAs1DForOutWhenUnconnected=off
  wires:
  Ground/1 -> Out/1

== system ASM_Traffic/ElectricalSystem/SignalInterface/ASMSignalInterface/signal_structure ==
  ASMSignalBus : Inport
  Battery_HV : BusSelector  OutputSignals=V_Bat[V],SOC_Bat[%],T_Bat[degC]
  Battery_LV : BusSelector  OutputSignals=V_Bat[V],SOC_Bat[%],T_Bat[degC]
  BusSelector_1 : BusSelector  OutputSignals=Battery_LV,Battery_HV,DCLink
  ContentID : Constant  Value=97540405
  DCLink : BusSelector  OutputSignals=V_DCLink[V]
  InfoBlock : Subsystem
      mask Display: fprintf('Structural changes of the signal bus require an update \nof the ''ASMSignalCollector'' block. \n\nTo start the update process double click the parent block.\n\n WARNING:\n During update this subsystem will be cleared completely')
  MDLD_DATA_CAPTURE : MDLD_Utils_lib/ModelDeskPlotInterface/DataCapture_Sfcn/MDLD_DATA_CAPTURE  inputPortWidth=7  measurementSignals=[0 0 0 0 0 0 0]  downsampling=1  samplingPeriod=SIM.StepSize.v  uuid=0  ASMProperties=struct('Name','mdld_data_capture','Version','1.0','Library','mdld_utils_lib')  startTriggerDelay=0  startTriggerLogic=0  startTriggerCount=0  startTriggerConditions=[0,0,0,0,0,0,0,0,0]  stopTriggerDelay=0  stopTriggerLogic=0  stopTriggerCount=0  stopTriggerConditions=[0,0,0,0,0,0,0,0,0]  ContentID_RefStruct=97540405
  SignalFilter : Mux  Inputs=7
  SignalFilterGain : Gain
  Terminator : Terminator
  wires:
  ASMSignalBus/1 -> BusSelector_1/1
  BusSelector_1/1 -> Battery_LV/1  "<Battery_LV>"
  BusSelector_1/2 -> Battery_HV/1  "<Battery_HV>"
  BusSelector_1/3 -> DCLink/1  "<DCLink>"
  ContentID/1 -> Terminator/1
  Battery_LV/1 -> SignalFilter/1  "<V_Bat[V]>"
  Battery_LV/2 -> SignalFilter/2  "<SOC_Bat[%]>"
  Battery_LV/3 -> SignalFilter/3  "<T_Bat[degC]>"
  Battery_HV/1 -> SignalFilter/4  "<V_Bat[V]>"
  Battery_HV/2 -> SignalFilter/5  "<SOC_Bat[%]>"
  Battery_HV/3 -> SignalFilter/6  "<T_Bat[degC]>"
  DCLink/1 -> SignalFilter/7  "<V_DCLink[V]>"
  SignalFilter/1 -> SignalFilterGain/1
  SignalFilterGain/1 -> MDLD_DATA_CAPTURE/1

== system ASM_Traffic/Engine/Control/SoftECU_Engine/SoftECU_Engine ==
  Trq_Driver_Des[Nm] : Inport
  Trq_Driver_Ind_Des[Nm] : Inport  Port=2
  Trq_Engine_Ind_Max[Nm] : Inport  Port=3
  Enable_Trq_Decrease_Fast_ESP[0|1] : Inport  Port=4
  Trq_Decrease_Request_Fast_ESP[Nm] : Inport  Port=5
  Enable_Trq_Increase_Fast_ESP[0|1] : Inport  Port=6
  Trq_Increase_Request_Fast_ESP[Nm] : Inport  Port=7
  Enable_Trq_Request_Extern1[0|1] : Inport  Port=8
  Trq_Request_Extern1[Nm] : Inport  Port=9
  Enable_Trq_Request_Extern2[0|1] : Inport  Port=10
  Trq_Request_Extern2[Nm] : Inport  Port=11
  Enable_n_Engine_Idle_Request[0|1] : Inport  Port=12
  n_Engine_Idle_Request[rpm] : Inport  Port=13
  n_Engine[rpm] : Inport  Port=14
  Pos_AccPedal_Driver[%] : Inport  Port=15
  Sw_Ignition[0Off|1On] : Inport  Port=16
  Sw_StarterReq[0Off|1On] : Inport  Port=17
  Reset[0|1] : Inport  Port=18
  Sw_CrankShaft_Reset[0Disabled|1Enabled] : Inport  Port=19
  Factor_Trq_Engine_Red[%] : Inport  Port=20
  Mode_StartButtonState[1Stim|2SoftECU] : Inport  Port=21
  State_StartButton[-1|0|1|2] : Inport  Port=22
  Trq_Request_ICE[Nm] : Inport  Port=23
  Vehicle_Topology[-2|-1|0|2] : Inport  Port=24
  ASMBUS_ENGINE_OPERATION : GotoTagVisibility  GotoTag=ASMBUS_ENGINE_OPERATION
  ASMBUS_ESP_FAST_TORQUE_SET : GotoTagVisibility  GotoTag=ASMBUS_ESP_FAST_TORQUE_SET
  ASMBUS_IDLE_SPEED_CONTROL : GotoTagVisibility  GotoTag=ASMBUS_IDLE_SPEED_CONTROL
  ASMBUS_SHIFT_TORQUE_SET : GotoTagVisibility  GotoTag=ASMBUS_SHIFT_TORQUE_SET
  ASMBUS_TORQUE_INTERVENTION : GotoTagVisibility  GotoTag=ASMBUS_TORQUE_INTERVENTION
  ASMSignalCollector : Subsystem
  Disable : Constant  Value=0  OutDataTypeStr=Inherit: Inherit via back propagation
  DisableReset : Subsystem
      mask Display: disp('DisableReset')
  ENGINE_OPERATION_BASIC : ASM_VehicleDynamics_lib/SoftECU/SoftECU_EngineBasic/ENGINE_OPERATION_BASIC  Tag=ASM_SUBCOMPONENT  Const_n_Engine_Min_EngineOn=MDL.SoftECU.EngineBasic.EngineOperation.Const_n_Engine_Min_EngineOn  Const_t_Max_Starter=MDL.SoftECU.EngineBasic.EngineOperation.Const_t_Max_Starter  Const_n_Engine_LowLim_Shutdown=MDL.SoftECU.EngineBasic.EngineOperation.Const_n_Engine_LowLim_Shutdown  Const_t_Shutdown=MDL.SoftECU.EngineBasic.EngineOperation.Const_t_Shutdown  StepSize=SIM.StepSize  ASMProperties=struct('Name','ENGINE_OPERATION_BASIC','Version','2.0','Library','ASM_VehicleDynamics_lib')  ASMInstanceName=engine_operation_basic  ASMInstanceID=1
  ESP_FAST_TORQUE_SET : ASM_VehicleDynamics_lib/SoftECU/SoftECU_EngineBasic/ESP_FAST_TORQUE_SET  Tag=ASM_SUBCOMPONENT  StepSize=SIM.StepSize  ASMProperties=struct('Name','ESP_FAST_TORQUE_SET','Version','3.0','Library','ASM_VehicleDynamics_lib')  ASMInstanceName=esp_fast_torque_set  ASMInstanceID=1
  IDLE_SPEED_CONTROL_ENGINE_BASIC : ASM_VehicleDynamics_lib/SoftECU/SoftECU_EngineBasic/IDLE_SPEED_CONTROL_ENGINE_BASIC  Tag=ASM_SUBCOMPONENT  Const_n_EngineIdle_Set=MDL.SoftECU.EngineBasic.Const_n_EngineIdle_Set  Const_P_Idle=MDL.SoftECU.EngineBasic.Const_P_Idle  Const_I_Idle=MDL.SoftECU.EngineBasic.Const_I_Idle  StepSize=SIM.StepSize  ASMProperties=struct('Name','IDLE_SPEED_CONTROL_ENGINE_BASIC','Version','5.0','Library','ASM_VehicleDynamics_lib')  ASMInstanceName=idle_speed_control_engine_basic  ASMInstanceID=1
  Memory : Memory
  Memory1 : Memory
  SHIFT_TORQUE_SET : ASM_VehicleDynamics_lib/SoftECU/SoftECU_EngineBasic/SHIFT_TORQUE_SET  Tag=ASM_SUBCOMPONENT  ASMProperties=struct('Name','SHIFT_TORQUE_SET','Version','2.0','Library','ASM_VehicleDynamics_lib')  ASMInstanceName=shift_torque_set  ASMInstanceID=1
  Sw_Intrv[0PosAcc|1Trq] : Constant  OutDataTypeStr=Inherit: Inherit via back propagation
  Switch : Switch  Criteria=u2 ~= 0  SaturateOnIntegerOverflow=off  InputSameDT=off
  Switch1 : Switch  Criteria=u2 ~= 0  SaturateOnIntegerOverflow=off  InputSameDT=off
  TORQUE_INTERVENTION_BASIC : ASM_VehicleDynamics_lib/SoftECU/SoftECU_EngineBasic/TORQUE_INTERVENTION_BASIC  Tag=ASM_SUBCOMPONENT  Map_Trq_Engine_Inv=MDL.SoftECU.EngineBasic.Map_Trq_Engine_Inv  StepSize=SIM.StepSize  ASMProperties=struct('Name','TORQUE_INTERVENTION_BASIC','Version','5.0','Library','ASM_VehicleDynamics_lib')  ASMInstanceName=torque_intervention_basic  ASMInstanceID=1
  Torque_Intervention_During_Gear_Shift : Subsystem
  Vehicle_Topology_Switch : Subsystem
  avoid_incomplete_trace2source : Subsystem
  avoid_incomplete_trace2source1 : Subsystem
  ASMSignalBus : Outport  VectorParamsAs1DForOutWhenUnconnected=off
  Sw_Engine_Dynamics_Fast[0|1] : Outport  Port=2  VectorParamsAs1DForOutWhenUnconnected=off
  Enable_Trq_Shift_Request[0|1] : Outport  Port=3  VectorParamsAs1DForOutWhenUnconnected=off
  Trq_Shift_Request[Nm] : Outport  Port=4  VectorParamsAs1DForOutWhenUnconnected=off
  Pos_AccPedal_Ctrl[%] : Outport  Port=5  VectorParamsAs1DForOutWhenUnconnected=off
  Pos_AccPedal_Driver_Des[%] : Outport  Port=6  VectorParamsAs1DForOutWhenUnconnected=off
  Sw_Starter[0Off|1On] : Outport  Port=7  VectorParamsAs1DForOutWhenUnconnected=off
  State_Engine[0|1|2|3|4] : Outport  Port=8  VectorParamsAs1DForOutWhenUnconnected=off
  n_Engine_Idle_Set[rpm] : Outport  Port=9  VectorParamsAs1DForOutWhenUnconnected=off
  tag scope: ASMBUS_ENGINE_OPERATION=scoped, ASMBUS_ESP_FAST_TORQUE_SET=scoped, ASMBUS_IDLE_SPEED_CONTROL=scoped, ASMBUS_SHIFT_TORQUE_SET=scoped, ASMBUS_TORQUE_INTERVENTION=scoped
  wires:
  avoid_incomplete_trace2source1/1(Out1) -> SHIFT_TORQUE_SET/1
  Trq_Driver_Ind_Des[Nm]/1 -> avoid_incomplete_trace2source1/1(In1)
  avoid_incomplete_trace2source/1(Out1) -> ESP_FAST_TORQUE_SET/1
  Enable_Trq_Decrease_Fast_ESP[0|1]/1 -> avoid_incomplete_trace2source/1(In1)
  State_StartButton[-1|0|1|2]/1 -> ENGINE_OPERATION_BASIC/6
  Mode_StartButtonState[1Stim|2SoftECU]/1 -> ENGINE_OPERATION_BASIC/5
  Trq_Engine_Ind_Max[Nm]/1 -> SHIFT_TORQUE_SET/3
  Factor_Trq_Engine_Red[%]/1 -> Torque_Intervention_During_Gear_Shift/1(Factor_Trq_Engine_Red[%]), SHIFT_TORQUE_SET/2
  Enable_Trq_Request_Extern1[0|1]/1 -> TORQUE_INTERVENTION_BASIC/3
  Trq_Request_Extern1[Nm]/1 -> TORQUE_INTERVENTION_BASIC/4
  Trq_Decrease_Request_Fast_ESP[Nm]/1 -> ESP_FAST_TORQUE_SET/2
  Enable_Trq_Increase_Fast_ESP[0|1]/1 -> ESP_FAST_TORQUE_SET/3
  Trq_Increase_Request_Fast_ESP[Nm]/1 -> ESP_FAST_TORQUE_SET/4
  ESP_FAST_TORQUE_SET/1 -> [ASMBUS_ESP_FAST_TORQUE_SET]
  Trq_Driver_Des[Nm]/1 -> ESP_FAST_TORQUE_SET/5
  ESP_FAST_TORQUE_SET/2 -> Sw_Engine_Dynamics_Fast[0|1]/1
  TORQUE_INTERVENTION_BASIC/1 -> [ASMBUS_TORQUE_INTERVENTION]
  ESP_FAST_TORQUE_SET/3 -> TORQUE_INTERVENTION_BASIC/1
  ESP_FAST_TORQUE_SET/4 -> TORQUE_INTERVENTION_BASIC/2
  ENGINE_OPERATION_BASIC/2 -> Sw_Starter[0Off|1On]/1
  ENGINE_OPERATION_BASIC/1 -> [ASMBUS_ENGINE_OPERATION]
  Vehicle_Topology_Switch/1(Pos_AccPedal_Driver[%]) -> Torque_Intervention_During_Gear_Shift/2(Pos_AccPedal_Driver[%]), Switch1/3, IDLE_SPEED_CONTROL_ENGINE_BASIC/2
  n_Engine_Idle_Request[rpm]/1 -> IDLE_SPEED_CONTROL_ENGINE_BASIC/7
  Enable_n_Engine_Idle_Request[0|1]/1 -> IDLE_SPEED_CONTROL_ENGINE_BASIC/6
  DisableReset/1(Reset[0|1]) -> ENGINE_OPERATION_BASIC/4
  Sw_StarterReq[0Off|1On]/1 -> Memory1/1
  SHIFT_TORQUE_SET/3 -> TORQUE_INTERVENTION_BASIC/8, Trq_Shift_Request[Nm]/1
  Reset[0|1]/1 -> ESP_FAST_TORQUE_SET/6, TORQUE_INTERVENTION_BASIC/11, IDLE_SPEED_CONTROL_ENGINE_BASIC/5, DisableReset/1(Reset_VehicleStates[0|1])
  IDLE_SPEED_CONTROL_ENGINE_BASIC/1 -> [ASMBUS_IDLE_SPEED_CONTROL]
  Sw_Ignition[0Off|1On]/1 -> Memory/1
  IDLE_SPEED_CONTROL_ENGINE_BASIC/3 -> Pos_AccPedal_Driver_Des[%]/1
  IDLE_SPEED_CONTROL_ENGINE_BASIC/2 -> Pos_AccPedal_Ctrl[%]/1
  n_Engine[rpm]/1 -> TORQUE_INTERVENTION_BASIC/10, IDLE_SPEED_CONTROL_ENGINE_BASIC/3, ENGINE_OPERATION_BASIC/3
  SHIFT_TORQUE_SET/2 -> Enable_Trq_Shift_Request[0|1]/1, Switch/3
  SHIFT_TORQUE_SET/1 -> [ASMBUS_SHIFT_TORQUE_SET]
  TORQUE_INTERVENTION_BASIC/2 -> IDLE_SPEED_CONTROL_ENGINE_BASIC/1
  Memory/1 -> IDLE_SPEED_CONTROL_ENGINE_BASIC/4, ENGINE_OPERATION_BASIC/1
  Memory1/1 -> ENGINE_OPERATION_BASIC/2
  Sw_CrankShaft_Reset[0Disabled|1Enabled]/1 -> DisableReset/2(Sw_CrankShaft_Reset[0Disabled|1Enabled])
  ASMSignalCollector/1(ASMSignalBus) -> ASMSignalBus/1
  ENGINE_OPERATION_BASIC/3 -> State_Engine[0|1|2|3|4]/1
  IDLE_SPEED_CONTROL_ENGINE_BASIC/4 -> n_Engine_Idle_Set[rpm]/1
  Disable/1 -> Switch/1
  Torque_Intervention_During_Gear_Shift/1(Pos_AccPedal[%]) -> Switch1/1
  Switch/1 -> TORQUE_INTERVENTION_BASIC/7
  Sw_Intrv[0PosAcc|1Trq]/1 -> Switch1/2, Switch/2
  Switch1/1 -> TORQUE_INTERVENTION_BASIC/9
  Pos_AccPedal_Driver[%]/1 -> Vehicle_Topology_Switch/2(Pos_AccPedal[%])
  Vehicle_Topology[-2|-1|0|2]/1 -> Vehicle_Topology_Switch/1(Vehicle_Topology[-2|-1|0|2])
  Enable_Trq_Request_Extern2[0|1]/1 -> Vehicle_Topology_Switch/3(Enable_Trq_Request_Extern2[0|1])
  Trq_Request_Extern2[Nm]/1 -> Vehicle_Topology_Switch/4(Trq_Request_Extern2[Nm])
  Trq_Request_ICE[Nm]/1 -> Vehicle_Topology_Switch/5(Trq_Request_ICE[Nm])
  Vehicle_Topology_Switch/2(Enable_Trq_Extern[0|1]) -> TORQUE_INTERVENTION_BASIC/5
  Vehicle_Topology_Switch/3(Trq_Request_Extern[Nm]) -> TORQUE_INTERVENTION_BASIC/6

== system ASM_Traffic/Engine/Control/UserInterface/ASMSignalBus_Control ==
  In : Inport
  Terminator_1 : Terminator
  tag scope: ASMBUS_Engine_Control=global
  wires:
  [ASMBUS_Engine_Control] -> Terminator_1/1
  In/1 -> [ASMBUS_Engine_Control]  "Control"

== system ASM_Traffic/Engine/Control/UserInterface/DISP_Control ==
  In : Inport
  Bus Selector2 : BusSelector  OutputSignals=Torque_Intervention.Enable_Trq_Request_Fast[0|1],Torque_Intervention.Enable_Trq_Request_Extern1[0|1],Torque_Intervention.Enable_Trq_Request_Extern2[0|1],Torque_Intervention.Enable_Trq_Request_Extern3[0|1],Torque_Intervention.Trq_Request_Fast[Nm],Torque_Intervention.Trq_Request_Extern1[Nm],Torque_Intervention.Trq_Request_Extern2[Nm],Torque_Intervention.Trq_Request_Extern3[Nm],Torque_Intervention.Pos_AccPedal_Request_Driver[%],Torque_Intervention.Pos_AccPedal_Request[%],EngineOperation.State_Engine[0|1|2|3|4],EngineOperation.Sw_Starter[0Off|1On]
  Enable_Trq_Request_Extern1[0|1] : Subsystem
      mask Display: disp('')
  Enable_Trq_Request_Extern2[0|1] : Subsystem
      mask Display: disp('')
  Enable_Trq_Request_Extern3[0|1] : Subsystem
      mask Display: disp('')
  Enable_Trq_Request_Fast[0|1] : Subsystem
      mask Display: disp('')
  Mux1 : Mux
  Mux2 : Mux  Inputs=2
  Mux3 : Mux
  Mux4 : Mux  Inputs=2
  Pos_AccPedal_Request[%] : Subsystem
      mask Display: disp('')
  Pos_AccPedal_Request_Driver[%] : Subsystem
      mask Display: disp('')
  SoftECU_Engine : Scope  NumInputPorts=4
      settings: TimeSpan=5  ActiveDisplayYMinimum=-42.03413  ActiveDisplayYMaximum=378.30719  DataLoggingMaxPoints=20000  DataLoggingDecimation=10
  State_Engine[0|1|2|3|4] : Subsystem
      mask Display: disp('')
  Sw_Starter[0|1] : Subsystem
      mask Display: disp('')
  Trq_Request_Extern1[Nm] : Subsystem
      mask Display: disp('')
  Trq_Request_Extern2[Nm] : Subsystem
      mask Display: disp('')
  Trq_Request_Extern3[Nm] : Subsystem
      mask Display: disp('')
  Trq_Request_Fast[Nm] : Subsystem
      mask Display: disp('')
  wires:
  In/1 -> Bus Selector2/1
  Bus Selector2/1 -> Enable_Trq_Request_Fast[0|1]/1(In1)  "<Enable_Trq_Request_Fast[0|1]>"
  Bus Selector2/2 -> Enable_Trq_Request_Extern1[0|1]/1(In1)  "<Enable_Trq_Request_Extern1[0|1]>"
  Bus Selector2/3 -> Enable_Trq_Request_Extern2[0|1]/1(In1)  "<Enable_Trq_Request_Extern2[0|1]>"
  Bus Selector2/4 -> Enable_Trq_Request_Extern3[0|1]/1(In1)  "<Enable_Trq_Request_Extern3[0|1]>"
  Bus Selector2/5 -> Trq_Request_Fast[Nm]/1(In1)  "<Trq_Request_Fast[Nm]>"
  Bus Selector2/6 -> Trq_Request_Extern1[Nm]/1(In1)  "<Trq_Request_Extern1[Nm]>"
  Bus Selector2/7 -> Trq_Request_Extern2[Nm]/1(In1)  "<Trq_Request_Extern2[Nm]>"
  Bus Selector2/8 -> Trq_Request_Extern3[Nm]/1(In1)  "<Trq_Request_Extern3[Nm]>"
  Bus Selector2/9 -> Pos_AccPedal_Request_Driver[%]/1(In1)  "<Pos_AccPedal_Request_Driver[%]>"
  Bus Selector2/10 -> Pos_AccPedal_Request[%]/1(In1)  "<Pos_AccPedal_Request[%]>"
  Bus Selector2/11 -> State_Engine[0|1|2|3|4]/1(In1)  "<State_Engine[0|1|2|3|4]>"
  Bus Selector2/12 -> Sw_Starter[0|1]/1(In1)  "<Sw_Starter[0Off|1On]>"
  Enable_Trq_Request_Fast[0|1]/1(Out1) -> Mux3/1
  Enable_Trq_Request_Extern1[0|1]/1(Out1) -> Mux3/2
  Enable_Trq_Request_Extern2[0|1]/1(Out1) -> Mux3/3
  Enable_Trq_Request_Extern3[0|1]/1(Out1) -> Mux3/4
  Trq_Request_Fast[Nm]/1(Out1) -> Mux1/1
  Trq_Request_Extern1[Nm]/1(Out1) -> Mux1/2
  Trq_Request_Extern2[Nm]/1(Out1) -> Mux1/3
  Trq_Request_Extern3[Nm]/1(Out1) -> Mux1/4
  Pos_AccPedal_Request_Driver[%]/1(Out1) -> Mux2/1
  Pos_AccPedal_Request[%]/1(Out1) -> Mux2/2
  Mux2/1 -> SoftECU_Engine/3
  State_Engine[0|1|2|3|4]/1(Out1) -> Mux4/1
  Sw_Starter[0|1]/1(Out1) -> Mux4/2
  Mux3/1 -> SoftECU_Engine/1
  Mux1/1 -> SoftECU_Engine/2
  Mux4/1 -> SoftECU_Engine/4

== system ASM_Traffic/Engine/Control/UserInterface/PAR_Control ==
  Termination : Constant  Value=0
  Out : Outport  VectorParamsAs1DForOutWhenUnconnected=off
  wires:
  Termination/1 -> Out/1

== system ASM_Traffic/Engine/Interface_In/ModelSignals/Enable_Trq_Decrease_Fast_ESP[0|1]_ ==
  In1 : Inport
  Gain : Gain  SaturateOnIntegerOverflow=on  OutDataTypeStr=Inherit: Same as input  ParamDataTypeStr=Inherit: Same as input
  Out1 : Outport  VectorParamsAs1DForOutWhenUnconnected=off
  wires:
  In1/1 -> Gain/1
  Gain/1 -> Out1/1

== system ASM_Traffic/Engine/Interface_In/ModelSignals/Enable_Trq_Increase_Fast_ESP[0|1]_ ==
  In1 : Inport
  Gain : Gain  SaturateOnIntegerOverflow=on  OutDataTypeStr=Inherit: Same as input  ParamDataTypeStr=Inherit: Same as input
  Out1 : Outport  VectorParamsAs1DForOutWhenUnconnected=off
  wires:
  In1/1 -> Gain/1
  Gain/1 -> Out1/1

== system ASM_Traffic/Engine/Interface_In/ModelSignals/Enable_Trq_Request_Extern1[0|1]_ ==
  In1 : Inport
  Gain : Gain  SaturateOnIntegerOverflow=on  OutDataTypeStr=Inherit: Same as input  ParamDataTypeStr=Inherit: Same as input
  Out1 : Outport  VectorParamsAs1DForOutWhenUnconnected=off
  wires:
  In1/1 -> Gain/1
  Gain/1 -> Out1/1

== system ASM_Traffic/Engine/Interface_In/ModelSignals/Enable_Trq_Request_Extern2[0|1]_ ==
  In1 : Inport
  Gain : Gain  SaturateOnIntegerOverflow=on  OutDataTypeStr=Inherit: Same as input  ParamDataTypeStr=Inherit: Same as input
  Out1 : Outport  VectorParamsAs1DForOutWhenUnconnected=off
  wires:
  In1/1 -> Gain/1
  Gain/1 -> Out1/1

== system ASM_Traffic/Engine/Interface_In/ModelSignals/Enable_n_Engine_Idle_Request[0|1]_ ==
  In1 : Inport
  Gain : Gain  SaturateOnIntegerOverflow=on  OutDataTypeStr=Inherit: Same as input  ParamDataTypeStr=Inherit: Same as input
  Out1 : Outport  VectorParamsAs1DForOutWhenUnconnected=off
  wires:
  Gain/1 -> Out1/1
  In1/1 -> Gain/1

== system ASM_Traffic/Engine/Interface_In/ModelSignals/Factor_Trq_Engine_Red[%]_ ==
  In1 : Inport
  Gain : Gain  SaturateOnIntegerOverflow=on  OutDataTypeStr=Inherit: Same as input  ParamDataTypeStr=Inherit: Same as input
  Out1 : Outport  VectorParamsAs1DForOutWhenUnconnected=off
  wires:
  In1/1 -> Gain/1
  Gain/1 -> Out1/1
